simulink model "dhwplant"  (R2026b)
settings: Solver=ode1  StopTime=120  FixedStep=0.01
values from neighbouring files (symbols this model uses):
  Cdhw = 4000    [init_params.m]
  cpw = 4186    [init_params.m]    (also in test_ch_low.m)
  ffgain = ffon*cpw/60*(Tdhwset-Tin)    (= 2093)    [init_params.m]    (also in testdhw.m = ffon*cpw/60*(Tdhwset-Tin))
  flowoff = 2.0    (= 2)    [init_params.m]
  flowon = 2.5    [init_params.m]
  Hoff = 3    [init_params.m]
  Hon = 3    [init_params.m]
  Kidhw = 110    [init_params.m]
  Kpdhw = 800    [init_params.m]
  Ktdhw = 3    [init_params.m]
  Qmaxdhw = Qmax    (= 24000)    [init_params.m]
  Qmindhw = Qmin    (= 2400)    [init_params.m]
  Tdhwset = 45    [init_params.m]    (also in testdhw.m = 35)
  tflow = 60    [init_params.m]
  Tin = 15    [init_params.m]    (also in testdhw.m = 25)
  topen = 5    [init_params.m]
  Tstart = 20    [init_params.m]
libraries: slpidlib x1
settings Model: Creator=Ogun Serif  LastModifiedBy=Ogun Serif

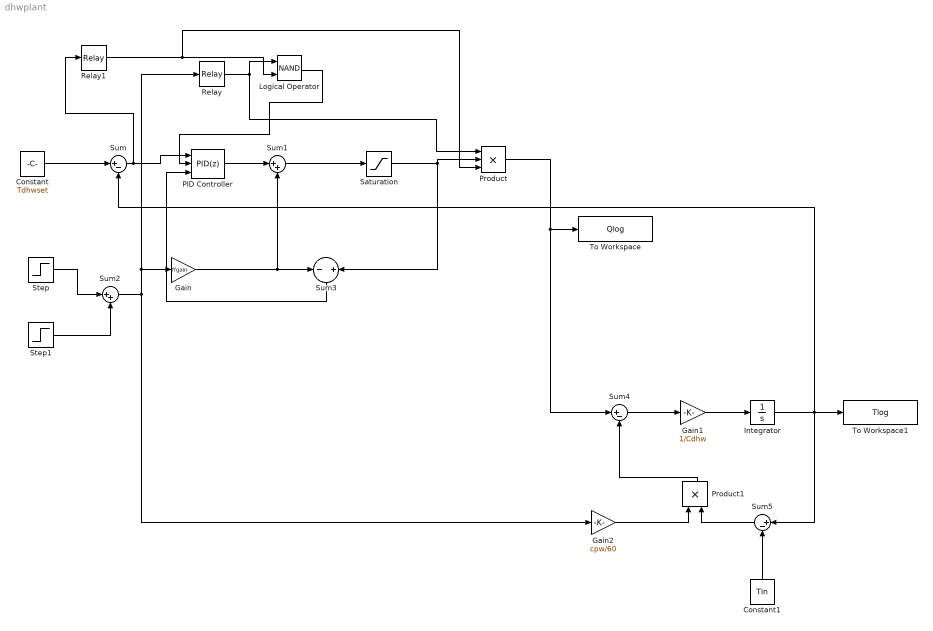
== system dhwplant ==
  Constant : Constant  Value=Tdhwset
  Constant1 : Constant  Value=Tin
  Gain : Gain  Gain=ffgain
  Gain1 : Gain  Gain=1/Cdhw
  Gain2 : Gain  Gain=cpw/60
  Integrator : Integrator  InitialCondition=Tstart
  Logical Operator : Logic  Operator=NAND  AllPortsSameDT=off  OutDataTypeStr=boolean
  PID Controller : slpidlib/PID Controller  Controller=PID  Form=Parallel  TimeDomain=Discrete-time  UseExternalTs=off  SampleTime=0.1  IntegratorMethod=Forward Euler  FilterMethod=Forward Euler  ControllerParametersSource=internal  P=Kpdhw  I=Kidhw  UseKiTs=off  D=0  UseExternalDerivativeSource=off  N=100  UseFilter=on  TunerSelectOption=Transfer Function Based (PID Tuner App)  InitialConditionSource=internal  InitialConditionForIntegrator=0  InitialConditionForFilter=0  DifferentiatorICPrevScaledInput=0  ExternalReset=level  TrackingMode=on  Kt=Ktdhw  LimitOutput=off  SatLimitsSource=internal  UpperSaturationLimit=inf  LowerSaturationLimit=-inf  LinearizeAsGain=on  AntiWindupMode=none  Kb=1  LimitIntegrator=off  UpperIntegratorSaturationLimit=inf  LowerIntegratorSaturationLimit=-inf  POutMin=[]  POutMax=[]  IOutMin=[]  IOutMax=[]  DOutMin=[]  DOutMax=[]  NOutMin=[]  NOutMax=[]  SumOutMin=[]  SumOutMax=[]  SaturationOutMin=[]  SaturationOutMax=[]  PParamMin=[]  PParamMax=[]  IParamMin=[]  IParamMax=[]  DParamMin=[]  DParamMax=[]  NParamMin=[]  NParamMax=[]  KbParamMin=[]  KbParamMax=[]  KtParamMin=[]  KtParamMax=[]  KbOutMin=[]  KbOutMax=[]  KtOutMin=[]  KtOutMax=[]  IntegratorOutMin=[]  IntegratorOutMax=[]  FilterOutMin=[]  FilterOutMax=[]  SumI1OutMin=[]  SumI1OutMax=[]  SumI2OutMin=[]  SumI2OutMax=[]  SumI3OutMin=[]  SumI3OutMax=[]  SumI4OutMin=[]  SumI4OutMax=[]  SumDOutMin=[]  SumDOutMax=[]  DifferentiatorOutMin=[]  DifferentiatorOutMax=[]  FilterDiffOutCoefMin=[]  FilterDiffOutCoefMax=[]  ReciprocalOutMin=[]  ReciprocalOutMax=[]  SumDenOutMin=[]  SumDenOutMax=[]  SumNumOutMin=[]  SumNumOutMax=[]  DivideOutMin=[]  DivideOutMax=[]  UdiffTsProdOutMin=[]  UdiffTsProdOutMax=[]  NTsProdOutMin=[]  NTsProdOutMax=[]  UintegralTsProdOutMin=[]  UintegralTsProdOutMax=[]  UngainTsProdOutMin=[]  UngainTsProdOutMax=[]  ClampingZeroOutDataTypeStr=Inherit: Inherit via back propagation  ClampingZeroOutMin=[]  ClampingZeroOutMax=[]  FilterDenConstantOutDataTypeStr=Inherit: Inherit via back propagation  FilterDenConstantOutMin=[]  FilterDenConstantOutMax=[]  PCopyOutDataTypeStr=Inherit: Inherit via back propagation  PCopyOutMin=[]  PCopyOutMax=[]  NCopyOutDataTypeStr=Inherit: Inherit via back propagation  NCopyOutMin=[]  NCopyOutMax=[]  IntegratorContinuousStateAttributes=''  IntegratorStateMustResolveToSignalObject=off  IntegratorRTWStateStorageClass=Auto  FilterContinuousStateAttributes=''  FilterStateMustResolveToSignalObject=off  FilterRTWStateStorageClass=Auto  ParallelPVariant=InternalParameters  IdealPVariant=Disabled  IVariant=InternalParameters  DVariant=InternalParameters  IntegratorVariant=Discrete  SatVariant=Disabled  AWVariant=Passthrough  PCopyVariant=Disabled  TRVariant=Enabled  FdbkBlocksVariant=Forward  IdealPFdbkVariant=Disabled  SatFdbkVariant=Disabled  DerivativeFilterVariant=ForwardEulerFilter  NVariant=InternalParameters  NCopyVariant=Disabled  FilterICVariant=InternalICsFilter  IntegratorICVariant=InternalICs  ExternalResetVariant=ExternalReset  TRSumVariant=TrackingMode  SumFdbkVariant=Disabled  SumVariant=Sum_PID  TsampFilterVariant=InternalTs  TsampNgainVariant=Passthrough  TsampIntegralVariant=Disabled_SignalSpec  ExternalSaturationOutDataTypeStr=Inherit: Same as second input  DerivativeSourceVariant=ErrorSignal  PreIntVariant=InternalPreInt
  Product : Product  Inputs=3
  Product1 : Product
  Relay : Relay  OnSwitchValue=flowon  OffSwitchValue=flowoff
  Relay1 : Relay  OnSwitchValue=Hon  OffSwitchValue=-Hoff
  Saturation : Saturate  UpperLimit=Qmaxdhw  LowerLimit=Qmindhw
  Step : Step  Time=topen  FinalValue=flowinit  SampleTime=0
  Step1 : Step  Time=tflow  FinalValue=flowfinal-flowinit  SampleTime=0
  Sum : Sum  Inputs=|+-
  Sum1 : Sum  Inputs=|++
  Sum2 : Sum  Inputs=|++
  Sum3 : Sum  Inputs=-|+
  Sum4 : Sum  Inputs=|+-
  Sum5 : Sum  Inputs=|+-
  To Workspace : ToWorkspace  VariableName=Qlog  SaveFormat=Timeseries  SampleTime=-1
  To Workspace1 : ToWorkspace  VariableName=Tlog  SaveFormat=Timeseries  SampleTime=-1
  wires:
  Constant/1 -> Sum/1
  Sum/1 -> PID Controller/1, Relay1/1
  PID Controller/1 -> Sum1/1
  Logical Operator/1 -> PID Controller/2
  Relay/1 -> Logical Operator/1, Product/1
  Sum1/1 -> Saturation/1
  Saturation/1 -> Sum3/2, Product/2
  Step/1 -> Sum2/1
  Step1/1 -> Sum2/2
  Sum2/1 -> Gain2/1, Relay/1, Gain/1
  Gain/1 -> Sum3/1, Sum1/2
  Product/1 -> Sum4/1, To Workspace/1
  Sum4/1 -> Gain1/1
  Gain1/1 -> Integrator/1
  Integrator/1 -> Sum/2, Sum5/1, To Workspace1/1
  Constant1/1 -> Sum5/2
  Sum5/1 -> Product1/2
  Gain2/1 -> Product1/1
  Sum3/1 -> PID Controller/3
  Product1/1 -> Sum4/2
  Relay1/1 -> Product/3, Logical Operator/2
